simulink model "XMED01_reference"  (R2025a)
settings: Solver=FixedStepDiscrete  StartTime=0  StopTime=12  FixedStep=0.002  RelTol=1e-3
undefined symbols (not defined in the file): airway_resistance, leak_fraction, obstruction_factor, obstruction_time, patient_compliance, target_insp_pressure
settings Model: Creator=SimuVerity Contributors  LastModifiedBy=SimuVerity Contributors

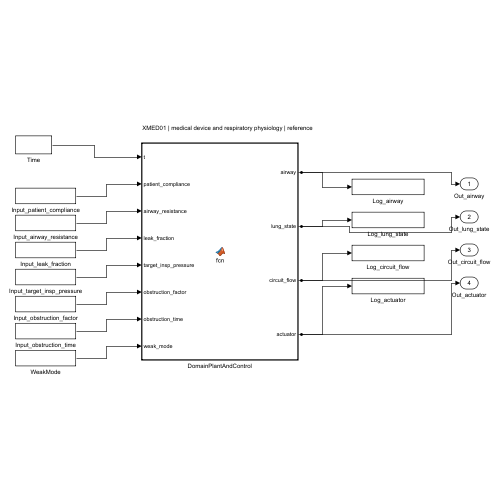
[thumbnail: Simulink's stored preview of the top-level diagram]
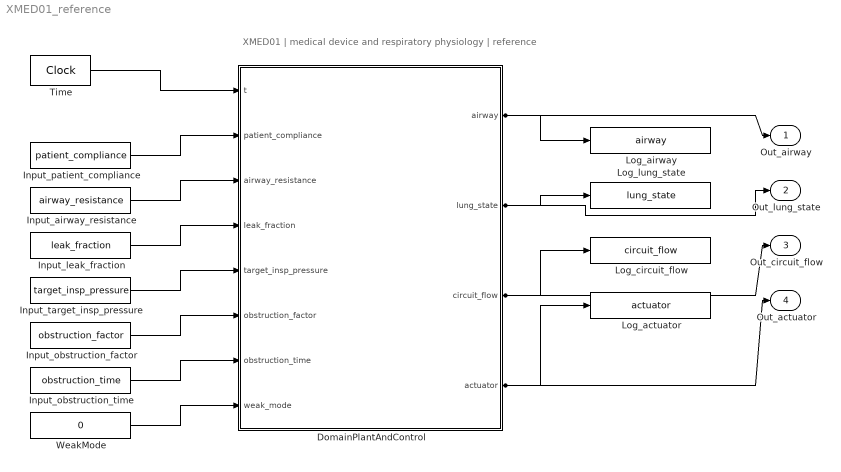
== system XMED01_reference ==
  note: XMED01 | medical device and respiratory physiology | reference
  DomainPlantAndControl : MATLAB Function  TreatAsAtomicUnit=on
  Input_airway_resistance : Constant  Value=airway_resistance
  Input_leak_fraction : Constant  Value=leak_fraction
  Input_obstruction_factor : Constant  Value=obstruction_factor
  Input_obstruction_time : Constant  Value=obstruction_time
  Input_patient_compliance : Constant  Value=patient_compliance
  Input_target_insp_pressure : Constant  Value=target_insp_pressure
  Log_actuator : ToWorkspace  VariableName=actuator  SaveFormat=Timeseries  SampleTime=-1
  Log_airway : ToWorkspace  VariableName=airway  SaveFormat=Timeseries  SampleTime=-1
  Log_circuit_flow : ToWorkspace  VariableName=circuit_flow  SaveFormat=Timeseries  SampleTime=-1
  Log_lung_state : ToWorkspace  VariableName=lung_state  SaveFormat=Timeseries  SampleTime=-1
  Time : DigitalClock  SampleTime=0.002
  WeakMode : Constant  Value=0
  Out_airway : Outport
  Out_lung_state : Outport  Port=2
  Out_circuit_flow : Outport  Port=3
  Out_actuator : Outport  Port=4
  wires:
  Time/1 -> DomainPlantAndControl/1(t)
  Input_patient_compliance/1 -> DomainPlantAndControl/2(patient_compliance)
  Input_airway_resistance/1 -> DomainPlantAndControl/3(airway_resistance)
  Input_leak_fraction/1 -> DomainPlantAndControl/4(leak_fraction)
  Input_target_insp_pressure/1 -> DomainPlantAndControl/5(target_insp_pressure)
  Input_obstruction_factor/1 -> DomainPlantAndControl/6(obstruction_factor)
  Input_obstruction_time/1 -> DomainPlantAndControl/7(obstruction_time)
  WeakMode/1 -> DomainPlantAndControl/8(weak_mode)
  DomainPlantAndControl/1(airway) -> Log_airway/1, Out_airway/1
  DomainPlantAndControl/2(lung_state) -> Log_lung_state/1, Out_lung_state/1
  DomainPlantAndControl/3(circuit_flow) -> Log_circuit_flow/1, Out_circuit_flow/1
  DomainPlantAndControl/4(actuator) -> Log_actuator/1, Out_actuator/1

== matlab function XMED01_reference/DomainPlantAndControl ==
  data: t input; airway output; patient_compliance input; airway_resistance input; leak_fraction input; target_insp_pressure input; obstruction_factor input; obstruction_time input; weak_mode input; lung_state output; circuit_flow output; actuator output
function [airway,lung_state,circuit_flow,actuator] = fcn(t,patient_compliance,airway_resistance,leak_fraction,target_insp_pressure,obstruction_factor,obstruction_time,weak_mode)
%#codegen
persistent V Paw integ alarmHold
dt=0.002; PEEP=5; supplyP=45;
if isempty(V)
    V=0; Paw=PEEP; integ=0; alarmHold=0;
end
phase=mod(t,3.0); insp=(phase<1.0);
target=PEEP; if insp, target=target_insp_pressure; end
event=(t>=obstruction_time && t<obstruction_time+1.0);
Reff=airway_resistance*(1+(obstruction_factor-1)*double(event));
Palv=PEEP+V/max(patient_compliance,0.005);
flow=(Paw-Palv)/max(Reff,1);
e=target-Paw;
if weak_mode<0.5
    if insp
        integ=min(max(integ+e*dt,-25),25);
        uin=min(max(0.110*e+0.045*integ+0.025,0),1);
        uout=min(max(-0.025*e,0),0.35);
    else
        uin=0; uout=min(max(0.075*(Paw-PEEP)+0.20,0),1);
        integ=0;
    end
else
    uin=0.43*double(insp); uout=0.38*double(~insp);
end
circuitCompliance=1/7;
leakFlow=(4/7)*leak_fraction*max(Paw,0)/18;
supplyFlow=(7.5/7)*uin*max(supplyP-Paw,0);
exhaustFlow=(10/7)*uout*max(Paw-PEEP,0);
dP=(supplyFlow-exhaustFlow-flow-leakFlow)/circuitCompliance;
Paw=Paw+dt*dP;
if Paw>35
    uin=0; uout=1; Paw=Paw-dt*30*(Paw-35);
end
V=max(V+dt*flow,0);
persistentErr=(insp && phase>0.40 && abs(e)>7) || (~insp && phase>1.40 && abs(e)>4);
bad=(Paw>32)||persistentErr;
if weak_mode<0.5
    if bad, alarmHold=0.8; else, alarmHold=max(alarmHold-dt,0); end
else
    alarmHold=0;
end
Palv=PEEP+V/max(patient_compliance,0.005);
flow=(Paw-Palv)/max(Reff,1);
leakFlow=(4/7)*leak_fraction*max(Paw,0)/18;
deliveredFlow=flow+leakFlow;
airway=[Paw,flow,V];
lung_state=Palv;
circuit_flow=[deliveredFlow,leakFlow];
actuator=[uin,uout,double(alarmHold>0)];
end
